simulink model "MotorGenerator1_Component_harness_model"  (R2023a)
settings: Solver=daessc  StartTime=0.0  StopTime=20  RelTol=1e-3  AbsTol=1e-3
PreLoadFcn:
  | MotorGenerator1_Component_harness_setup
undefined symbols (not defined in the file or in its folder): batteryHighVoltage, initial, Minus, motorGenerator1, Plus
libraries: fl_lib x24, nesl_utility x11, sdl_lib x3
settings Model: Creator=isaacito  LastModifiedBy=isaacito
settings SolverCC: AutoScaleAbsTol=off  AlgebraicLoopSolver=TrustRegion
settings OptimizationCC: ReuseModelBlockBuffer=off
settings DebuggingCC: UnconnectedInputMsg=warning  UnconnectedOutputMsg=warning  UnconnectedLineMsg=warning  SymbolicDimsDataTypeCodeGenerationDiagnostic=none
settings ModelReferenceCC: EnableRefExpFcnMdlSchedulingChecks=on
settings SFSimCC: CustomCodeUndefinedFunction=UseInterfaceOnly
settings RTWCC: DLArmComputeVersion=19.05
settings SimscapeCC: SimscapeLogType=all  SimscapeLogSimulationStatistics=on  SimscapeLogLimitData=off  SimscapeLogDataHistory=10000

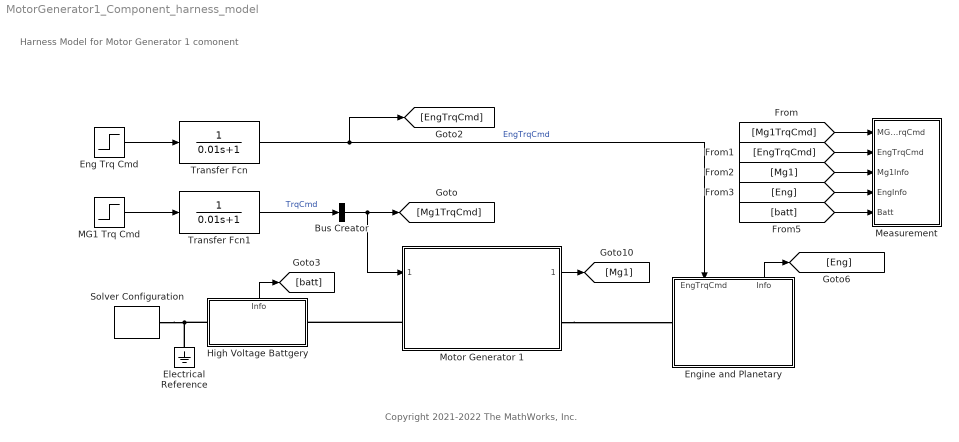
== system MotorGenerator1_Component_harness_model ==
  note: Harness Model for Motor Generator 1 comonent
  note: Copyright 2021-2022 The MathWorks, Inc.
  Bus Creator : BusCreator  Inputs=1
  Electrical Reference : fl_lib/Electrical/Electrical Elements/Electrical Reference
  Eng Trq Cmd : Step  Time=10  Before=100  After=0  SampleTime=0
      settings: AttributesFormatString=|
      | Before %<Before>
      | Time %<Time>
      | After %<After>
  Engine and Planetary : Subsystem
      settings: PortSchema="{\"entries\":[{\"content\":{\"sides\":[{\"content\":{\"connectorIds\":[\"LConn1\"]},\"type\":\"ConnectorPlacement.EquallySpacedRectSide\",\"uuid\":\"98e473f2-6fb6-4bf2-93a0-47b50a56d31a\"},{\"content\":{\"connectorIds\":[],\"side\":\"RIGHT\"},\"type\":\"ConnectorPlacement.EquallySpacedRectSide\",\"uuid\":\"e7c78de6-faab-4a88-b22a-7c9a139264de\"},{\"content\":{\"connectorIds\":[\"In1\",\"Out1\"],\"side\":\"TOP\"},\"type\":\"ConnectorPlacement.EquallySpacedRectSide\",\"uuid\":\"45493563-c3b6-4270-8bd2-a782db83b07f\"}]},\"type\":\"ConnectorPlacement.EquallySpacedConnector\",\"uuid\":\"120a86e3-ef09-4ca7-b56f-7271bd8d5896\"}],\"packageUris\":[\"http://schema.mathworks.com/mf0/Connector/R2020b\"],\"version\":\"1.0\"}"
  High Voltage Battgery : Subsystem
      settings: PortSchema="{\"entries\":[{\"content\":{\"sides\":[{\"content\":{\"connectorIds\":[\"LConn1\"]},\"type\":\"ConnectorPlacement.EquallySpacedRectSide\",\"uuid\":\"8acd7e9a-bb08-4de6-aa14-0989ebba81b9\"},{\"content\":{\"connectorIds\":[\"RConn1\"],\"side\":\"RIGHT\"},\"type\":\"ConnectorPlacement.EquallySpacedRectSide\",\"uuid\":\"f80e1afc-966f-4d6b-84f9-f0b60dd6f20c\"},{\"content\":{\"connectorIds\":[\"Out1\"],\"side\":\"TOP\"},\"type\":\"ConnectorPlacement.EquallySpacedRectSide\",\"uuid\":\"52ccb2b1-bd5e-4dcb-b9b6-0ef03b912c33\"}]},\"type\":\"ConnectorPlacement.EquallySpacedConnector\",\"uuid\":\"b55f48a4-f283-4a77-8513-99b31abb285a\"}],\"packageUris\":[\"http://schema.mathworks.com/mf0/Connector/R2020b\"],\"version\":\"1.0\"}"
  MG1 Trq Cmd : Step  Time=15  After=-5  SampleTime=0
      settings: AttributesFormatString=|
      | Before %<Before>
      | Time %<Time>
      | After %<After>
  Measurement : Subsystem
  Motor Generator 1 : Subsystem  ReferencedSubsystem=MotorDriveUnit_refsub_Basic  torque_max=motorGenerator1.trqMax_Nm  Value=motorGenerator1.powerMax_kW  Tc=motorGenerator1.responseTime_s  eff=motorGenerator1.efficiency_pct  w_eff=motorGenerator1.spd_eff_rpm  T_eff=motorGenerator1.trq_eff_Nm  thermal_mass=motorGenerator1.thermalMass_J_perK  temperature=initial.MG1_Temperature_K  k=motorGenerator1.dampSpringStiffness_Nm_per_rad  mu_visc=motorGenerator1.dampSpringFriction_Nm_per_rpm  w_tol=smoothing.MG1_dampSpringVelTol_rpm  T=initial.MG1_AirTemp_K
      settings: PortSchema="{\"entries\":[{\"content\":{\"sides\":[{\"content\":{\"connectorIds\":[\"In1\",\"LConn1\"]},\"type\":\"ConnectorPlacement.EquallySpacedRectSide\",\"uuid\":\"02d16a10-ccfb-4288-a5a1-1144159c5ca2\"},{\"content\":{\"connectorIds\":[\"Out1\",\"LConn2\"],\"side\":\"RIGHT\"},\"type\":\"ConnectorPlacement.EquallySpacedRectSide\",\"uuid\":\"b2601986-efe5-4f5e-bd54-3f5cb03e9252\"},{\"content\":{\"side\":\"TOP\"},\"type\":\"ConnectorPlacement.EquallySpacedRectSide\",\"uuid\":\"248805f0-4416-4f49-8b0b-c2d3fe77e89e\"}]},\"type\":\"ConnectorPlacement.EquallySpacedConnector\",\"uuid\":\"35449164-35fe-478e-9b2e-66e853caa6da\"}],\"packageUris\":[\"http://schema.mathworks.com/mf0/Connector/R2020b\"],\"version\":\"1.0\"}"
  Solver Configuration : nesl_utility/Solver Configuration  PhysicalDomain=network_engine_domain  SubClassName=solver  LeftPortType=input  RightPortType=generic  Tones=[]  Harmonics=[]  SimulateNoise=off  Profile=off  UseLocalSampling=off  EnableSwitchedLinearOptims=on  FrequencyDomain=off  UseCCode=off  RelTol=0.001  AbsTol=1e-06  MinStep=1e-09  ToWorkspace=off  RevertToSquareIcSolve=off  NumHomotopyIterations=100  PhasorMode=off  PhasorModeNumHarmonics=1  ConsistencySolver=NEWTON_FTOL  IndexReductionMethod=DerivativeReplacement  DoDC=off  ResidualTolerance=1e-09  ConsistencyTolSource=GLOBAL  ConsistencyAbsTol=0.001  ConsistencyRelTol=0.001  ConsistencyTolFactor=0.001  UseLocalSolver=off  LocalSolverChoice=NE_BACKWARD_EULER_ADVANCER  ResolveIndetEquations=on  FunctionEvalNumThread=1  LocalSolverSampleTime=0.001  DoFixedCost=off  MaxNonlinIter=3  MaxModeIter=2  ComputeImpulses=off  ImpulseIterations=2  LinearAlgebra=auto  LinearAlgebraNumThread=0  EquationFormulation=NE_TIME_EF  DelaysMemoryBudget=1024  AutomaticFiltering=on  FilteringTimeConstant=0.001  PartitionStorageMethod=AS_NEEDED  PartitionMemoryBudget=1024  PartitionMethod=ROBUST
      settings: AttributesFormatString=Local solver %<UseLocalSolver>
  Transfer Fcn : TransferFcn  Denominator=[0.01 1]
  Transfer Fcn1 : TransferFcn  Denominator=[0.01 1]
  wires:
  Motor Generator 1/1 -> [Mg1]
  High Voltage Battgery/1(Info) -> [batt]
  Engine and Planetary/1(Info) -> [Eng]
  Eng Trq Cmd/1 -> Transfer Fcn/1
  [Mg1] -> Measurement/3(Mg1Info)
  [Eng] -> Measurement/4(EngInfo)
  [batt] -> Measurement/5(Batt)
  [Mg1TrqCmd] -> Measurement/1(MG1TrqCmd)
  [EngTrqCmd] -> Measurement/2(EngTrqCmd)
  Bus Creator/1 -> Motor Generator 1/1, [Mg1TrqCmd]
  Transfer Fcn/1 -> [EngTrqCmd], Engine and Planetary/1(EngTrqCmd)  "EngTrqCmd"
  Transfer Fcn1/1 -> Bus Creator/1  "TrqCmd"
  MG1 Trq Cmd/1 -> Transfer Fcn1/1
  connections:
  Solver Configuration/RConn1 -- Electrical Reference/LConn1 -- High Voltage Battgery/LConn1
  Motor Generator 1/LConn1 -- High Voltage Battgery/RConn1
  Motor Generator 1/LConn2 -- Engine and Planetary/LConn1

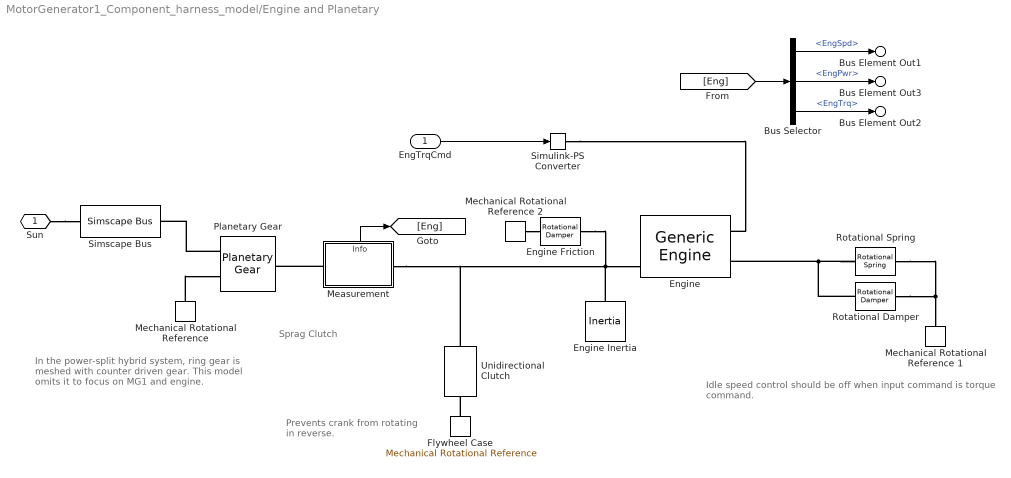
== system MotorGenerator1_Component_harness_model/Engine and Planetary ==
  note: Idle speed control should be off
      | when input command is torque command.
  note: Prevents crank from
      | rotating in reverse.
  note: In the power-split hybrid system,
      | ring gear is meshed with
      | counter driven gear.
      | This model omits it to focus on
      | MG1 and engine.
  note: Sprag Clutch
  EngTrqCmd : Inport
  Bus Selector : BusSelector  OutputSignals=EngSpd,EngPwr,EngTrq
  Engine : sdl_lib/Engines & Motors/Generic Engine  input_type=sdl.enum.GenericEngineInputType.TorqueCommand  model_parameterization=sdl.enum.engineParameterization.polynomial  engine_type=sdl.enum.engineType.Generic  Trq_max=145 N*m  w_Trq_max=3500 rpm  P_max=75 kW  w_P_max=7500 rpm  w_max=7000 rpm  w_min=500 rpm  w_tab=[500, 1000, 2000, 3000, 4300, 5000, 6000, 7000] rpm  trq_tab=[250, 280, 330, 360, 380, 370, 350, 310] N*m  pwr_tab=[10, 30, 70, 110, 165, 190, 220, 230] kW  interp_method=simscape.enum.interpolation.linear  w_thr=100 rpm  model_inertia=sdl.enum.model_inertia.off  inertia=1 kg*m^2  initial_velocity=800 rpm  model_time_constant=sdl.enum.lagOffOn.on  time_constant=0.1 s  initial_normalized_throttle=0  fc_model=sdl.enum.fuel_consumption_model.FuelOff  fc_per_rev=25 mg/rev  fc_w_tab=[1000, 2000, 3000, 4000, 5000, 6000] rpm  fc_trq_tab=[0, 80, 160, 200, 240, 320, 360, 400] N*m  fc_tab=[.5, .9, 1.4, 1.6, 1.9, 2.7, 3.4, 4.4; 1, 1.7, 2.7, 3.1, 3.6, 5, 6, 7.4; 1.4, 2.7, 4, 4.8, 5.6, 7.5, 8.5, 10.5; 2, 3.6, 5.8, 6.7, 8, 10.4, 11.7, 13.3; 2.5, 4.8, 7.9, 9.4, 10.8, 14, 16.2, 18.6; 3.1, 6, 10.3, 11.9, 13.8, 18.4, 22, 26.5] g/s  bmep_tab=[0, 250, 500, 625, 750, 1000, 1150, 1250] kPa  bsfc_tab=[410, 380, 300, 280, 270, 290, 320, 380; 410, 370, 290, 270, 260, 270, 285, 320; 415, 380, 290, 275, 265, 270, 270, 300; 420, 390, 310, 290, 285, 280, 280, 285; 430, 410, 340, 320, 310, 300, 310, 320; 450, 430, 370, 340, 330, 330, 350, 380] g/(hr*kW)  fc_interp_method=simscape.enum.interpolation.linear  displaced_volume=400 cm^3  rev_per_cycle=2  idle_speed=false  idle_speed_reference=1000 rpm  tau_controller=0.1 s  idle_w_thr=1 rpm  redline=false  redline_speed=5000 rpm  tau_redline=1 s  redline_w_thr=1 rpm
      settings: InternalSimscapePortConfiguration="{\"Bottom\":[],\"Left\":[{\"id\":\"TrqCmd\",\"label\":\"Trq\",\"type\":\"input\"},{\"id\":\"B\",\"label\":\"B\",\"type\":\"foundation.mechanical.rotational.rotational\"}],\"Right\":[{\"id\":\"P\",\"label\":\"P\",\"type\":\"output\"},{\"id\":\"FC\",\"label\":\"FC\",\"type\":\"output\"},{\"id\":\"F\",\"label\":\"F\",\"type\":\"foundation.mechanical.rotational.rotational\"}],\"Top\":[]}"
  Engine Friction : fl_lib/Mechanical/Rotational Elements/Rotational Damper  D=0.02 m*N/rpm  w_specify=off  w_priority=None  w=0 rad/s  w_nominal_specify=off  w_nominal_unit=rad/s  w_nominal_value=1  t_specify=off  t_priority=None  t=0 N*m  t_nominal_specify=off  t_nominal_unit=N*m  t_nominal_value=1
  Engine Inertia : fl_lib/Mechanical/Rotational Elements/Inertia  inertia=0.02 kg*m^2  num_ports=foundation.enum.numPorts2.one  w_specify=on  w_priority=High  w=initial.engine_speed_rpm rpm  w_nominal_specify=off  w_nominal_unit=rad/s  w_nominal_value=1  t_specify=off  t_priority=None  t=0 N*m  t_nominal_specify=off  t_nominal_unit=N*m  t_nominal_value=1
      settings: AttributesFormatString=|
      | %<inertia> (%<inertia_unit>)
      | %<w> (%<w_unit>)
      | Priority: %<w_priority>
  Flywheel Case : fl_lib/Mechanical/Rotational Elements/Mechanical Rotational Reference
  Measurement : Subsystem
      settings: PortSchema="{\"entries\":[{\"content\":{\"sides\":[{\"content\":{\"connectorIds\":[\"LConn1\"]},\"type\":\"ConnectorPlacement.EquallySpacedRectSide\",\"uuid\":\"98e473f2-6fb6-4bf2-93a0-47b50a56d31a\"},{\"content\":{\"connectorIds\":[\"RConn1\"],\"side\":\"RIGHT\"},\"type\":\"ConnectorPlacement.EquallySpacedRectSide\",\"uuid\":\"e7c78de6-faab-4a88-b22a-7c9a139264de\"},{\"content\":{\"connectorIds\":[\"Out1\"],\"side\":\"TOP\"},\"type\":\"ConnectorPlacement.EquallySpacedRectSide\",\"uuid\":\"45493563-c3b6-4270-8bd2-a782db83b07f\"}]},\"type\":\"ConnectorPlacement.EquallySpacedConnector\",\"uuid\":\"120a86e3-ef09-4ca7-b56f-7271bd8d5896\"}],\"packageUris\":[\"http://schema.mathworks.com/mf0/Connector/R2020b\"],\"version\":\"1.0\"}"
  Mechanical Rotational Reference : fl_lib/Mechanical/Rotational Elements/Mechanical Rotational Reference
  Mechanical Rotational Reference 1 : fl_lib/Mechanical/Rotational Elements/Mechanical Rotational Reference
  Mechanical Rotational Reference 2 : fl_lib/Mechanical/Rotational Elements/Mechanical Rotational Reference
  Planetary Gear : sdl_lib/Gears/Planetary Gear  rs_ratio=78/30  friction_model=sdl.enum.gear_friction.constant  efficiency=[0.98 0.98]  temperature_TLU=[280, 300, 320] K  efficiency_sp_TLU=[.95, .9, .85]  efficiency_rp_TLU=[.95, .9, .85]  pwr_thr=[10 10] W  mu_visc=[0.001 0.001] m*N/rpm  model_inertia=simscape.enum.onoff.on  planet_inertia=0.001 kg*m^2  thermal_mass=50 J/K  T_init=300 K
  Rotational Damper : fl_lib/Mechanical/Rotational Elements/Rotational Damper  D=100 kN*m/rpm  w_specify=off  w_priority=None  w=0 rad/s  w_nominal_specify=off  w_nominal_unit=rad/s  w_nominal_value=1  t_specify=off  t_priority=None  t=0 N*m  t_nominal_specify=off  t_nominal_unit=N*m  t_nominal_value=1
  Rotational Spring : fl_lib/Mechanical/Rotational Elements/Rotational Spring  spr_rate=1 kN*m/rad  w_specify=off  w_priority=None  w=0 rad/s  w_nominal_specify=off  w_nominal_unit=rad/s  w_nominal_value=1  t_specify=off  t_priority=None  t=0 N*m  t_nominal_specify=off  t_nominal_unit=N*m  t_nominal_value=1  phi_specify=on  phi_priority=Low  phi=0 rad  phi_nominal_specify=off  phi_nominal_unit=rad  phi_nominal_value=1
      settings: AttributesFormatString=Deformation priority: %<phi_priority>
  Simscape Bus : SimscapeBus  HierarchyStrings=AngSpd  ConnectionType=Bus: Bus_Rotational
  Simulink-PS Converter : nesl_utility/Simulink-PS Converter  PhysicalDomain=network_engine_domain  SubClassName=ps_input  LeftPortType=input  RightPortType=output  PseudoPeriodic=off  Frequencies=[]  NoiseDistribution=none  NoiseParameters=[]  Unit=N*m  AffineConversion=off  FilteringAndDerivatives=provide  SimscapeFilterOrder=1  InputFilterTimeConstant=0.001  UdotUserProvided=0
  Unidirectional Clutch : sdl_lib/Clutches/Unidirectional Clutch  transmission_direction=2  initial_state_locked=sdl.enum.initial_lock.unlocked
      settings: AttributesFormatString=%<initial_state_locked>  InternalSimscapePortConfiguration="{\"Bottom\":[],\"Left\":[{\"id\":\"H\",\"label\":\"H\",\"type\":\"foundation.mechanical.rotational.rotational\"}],\"Right\":[{\"id\":\"R\",\"label\":\"R\",\"type\":\"foundation.mechanical.rotational.rotational\"}],\"Top\":[]}"
  Sun : PMIOPort  Side=Left
  Bus Element Out1 : Outport  PortName=Info  Element=EngSpd
      settings: AttributesFormatString=%<Unit>
  Bus Element Out3 : Outport  PortName=Info  Element=EngPwr
      settings: AttributesFormatString=%<Unit>
  Bus Element Out2 : Outport  PortName=Info  Element=EngTrq
      settings: AttributesFormatString=%<Unit>
  wires:
  Measurement/1(Info) -> [Eng]
  [Eng] -> Bus Selector/1
  Bus Selector/1 -> Bus Element Out1/1  "<EngSpd>"
  Bus Selector/2 -> Bus Element Out3/1  "<EngPwr>"
  Bus Selector/3 -> Bus Element Out2/1  "<EngTrq>"
  EngTrqCmd/1 -> Simulink-PS Converter/1
  connections:
  Planetary Gear/RConn2 -- Simscape Bus/LConn1
  Sun/RConn1 -- Simscape Bus/RConn1
  Flywheel Case/LConn1 -- Unidirectional Clutch/RConn1
  Rotational Spring/RConn1 -- Rotational Damper/RConn1 -- Mechanical Rotational Reference 1/LConn1
  Rotational Spring/LConn1 -- Engine/LConn2 -- Rotational Damper/LConn1
  Mechanical Rotational Reference 2/LConn1 -- Engine Friction/RConn1
  Engine Friction/LConn1 -- Unidirectional Clutch/LConn1 -- Measurement/RConn1 -- Engine Inertia/LConn1 -- Engine/RConn3
  Measurement/LConn1 -- Planetary Gear/LConn1
  Mechanical Rotational Reference/LConn1 -- Planetary Gear/RConn1
  Simulink-PS Converter/RConn1 -- Engine/LConn1

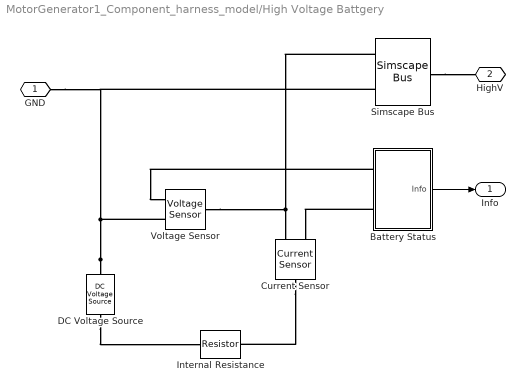
== system MotorGenerator1_Component_harness_model/High Voltage Battgery ==
  Battery Status : Subsystem
  Current Sensor : fl_lib/Electrical/Electrical Sensors/Current Sensor
  DC Voltage Source : fl_lib/Electrical/Electrical Sources/DC Voltage Source  v0=batteryHighVoltage.voltage_V V
      settings: AttributesFormatString=%<v0> [%<v0_unit>]
  Internal Resistance : fl_lib/Electrical/Electrical Elements/Resistor  R=batteryHighVoltage.internal_R_Ohm Ohm  i_specify=off  i_priority=High  i=0 A  i_nominal_specify=off  i_nominal_unit=A  i_nominal_value=1  v_specify=off  v_priority=High  v=0 V  v_nominal_specify=off  v_nominal_unit=V  v_nominal_value=1
      settings: AttributesFormatString=%<R> [%<R_unit>]
  Simscape Bus : SimscapeBus  HierarchyStrings=Plus;Minus  ConnectionType=Bus: Bus_HighVoltage
      settings: AttributesFormatString=%<ConnectionType>
  Voltage Sensor : fl_lib/Electrical/Electrical Sensors/Voltage Sensor
  GND : PMIOPort  Side=Left
  HighV : PMIOPort  Port=2  Side=Right
  Info : Outport
  wires:
  Battery Status/1(Info) -> Info/1
  connections:
  DC Voltage Source/RConn1 -- Simscape Bus/LConn2 -- GND/RConn1 -- Voltage Sensor/RConn2
  Simscape Bus/LConn1 -- Voltage Sensor/LConn1 -- Current Sensor/RConn2
  Battery Status/LConn2 -- Current Sensor/RConn1
  Simscape Bus/RConn1 -- HighV/RConn1
  Current Sensor/LConn1 -- Internal Resistance/RConn1
  DC Voltage Source/LConn1 -- Internal Resistance/LConn1
  Battery Status/LConn1 -- Voltage Sensor/RConn1

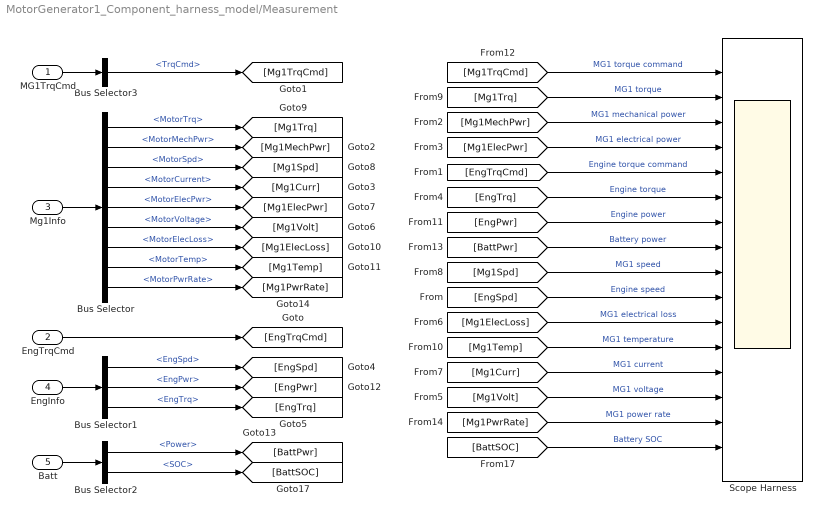
== system MotorGenerator1_Component_harness_model/Measurement ==
  MG1TrqCmd : Inport
  EngTrqCmd : Inport  Port=2
  Mg1Info : Inport  Port=3
  EngInfo : Inport  Port=4
  Batt : Inport  Port=5
  Bus Selector : BusSelector  OutputSignals=MotorTrq,MotorMechPwr,MotorSpd,MotorCurrent,MotorElecPwr,MotorVoltage,MotorElecLoss,MotorTemp,MotorPwrRate
  Bus Selector1 : BusSelector  OutputSignals=EngSpd,EngPwr,EngTrq
  Bus Selector2 : BusSelector  OutputSignals=Power,SOC
  Bus Selector3 : BusSelector  OutputSignals=TrqCmd
  Scope Harness : Scope  NumInputPorts=16
  wires:
  EngInfo/1 -> Bus Selector1/1
  Mg1Info/1 -> Bus Selector/1
  EngTrqCmd/1 -> [EngTrqCmd]
  Batt/1 -> Bus Selector2/1
  Bus Selector/1 -> [Mg1Trq]  "<MotorTrq>"
  Bus Selector/2 -> [Mg1MechPwr]  "<MotorMechPwr>"
  Bus Selector/3 -> [Mg1Spd]  "<MotorSpd>"
  Bus Selector/4 -> [Mg1Curr]  "<MotorCurrent>"
  Bus Selector/5 -> [Mg1ElecPwr]  "<MotorElecPwr>"
  Bus Selector/6 -> [Mg1Volt]  "<MotorVoltage>"
  Bus Selector/7 -> [Mg1ElecLoss]  "<MotorElecLoss>"
  Bus Selector/8 -> [Mg1Temp]  "<MotorTemp>"
  Bus Selector1/1 -> [EngSpd]  "<EngSpd>"
  Bus Selector1/2 -> [EngPwr]  "<EngPwr>"
  Bus Selector1/3 -> [EngTrq]  "<EngTrq>"
  Bus Selector2/1 -> [BattPwr]  "<Power>"
  Bus Selector2/2 -> [BattSOC]  "<SOC>"
  [Mg1TrqCmd] -> Scope Harness/1  "MG1 torque command"
  [Mg1Trq] -> Scope Harness/2  "MG1 torque"
  [Mg1MechPwr] -> Scope Harness/3  "MG1 mechanical power"
  [Mg1ElecPwr] -> Scope Harness/4  "MG1 electrical power"
  [EngTrqCmd] -> Scope Harness/5  "Engine torque command"
  [EngTrq] -> Scope Harness/6  "Engine torque"
  [EngPwr] -> Scope Harness/7  "Engine power"
  [BattPwr] -> Scope Harness/8  "Battery power"
  [Mg1Spd] -> Scope Harness/9  "MG1 speed"
  [EngSpd] -> Scope Harness/10  "Engine speed"
  [Mg1ElecLoss] -> Scope Harness/11  "MG1 electrical loss"
  [Mg1Temp] -> Scope Harness/12  "MG1 temperature"
  [Mg1Curr] -> Scope Harness/13  "MG1 current"
  [Mg1Volt] -> Scope Harness/14  "MG1 voltage"
  [BattSOC] -> Scope Harness/16  "Battery SOC"
  MG1TrqCmd/1 -> Bus Selector3/1
  Bus Selector3/1 -> [Mg1TrqCmd]  "<TrqCmd>"
  Bus Selector/9 -> [Mg1PwrRate]  "<MotorPwrRate>"
  [Mg1PwrRate] -> Scope Harness/15  "MG1 power rate"

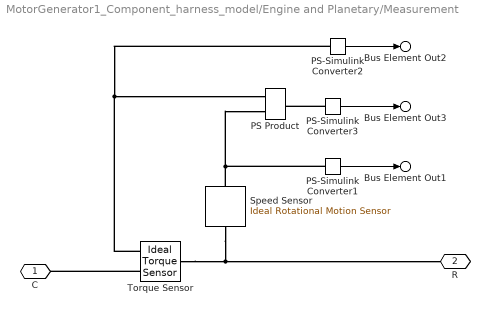
== system MotorGenerator1_Component_harness_model/Engine and Planetary/Measurement ==
  PS Product : fl_lib/Physical Signals/Functions/PS Product
  PS-Simulink Converter1 : nesl_utility/PS-Simulink Converter  PhysicalDomain=network_engine_domain  SubClassName=ps_output  LeftPortType=input  RightPortType=output  PseudoPeriodic=off  Frequencies=[]  VectorFormat=1-D array  Unit=rpm  AffineConversion=off
  PS-Simulink Converter2 : nesl_utility/PS-Simulink Converter  PhysicalDomain=network_engine_domain  SubClassName=ps_output  LeftPortType=input  RightPortType=output  PseudoPeriodic=off  Frequencies=[]  VectorFormat=1-D array  Unit=N*m  AffineConversion=off
  PS-Simulink Converter3 : nesl_utility/PS-Simulink Converter  PhysicalDomain=network_engine_domain  SubClassName=ps_output  LeftPortType=input  RightPortType=output  PseudoPeriodic=off  Frequencies=[]  VectorFormat=1-D array  Unit=kW  AffineConversion=off
  Speed Sensor : fl_lib/Mechanical/Mechanical Sensors/Ideal Rotational Motion Sensor  reference=foundation.enum.MeasurementReference.absolute  acceleration_port=false  velocity_port=true  position_port=false  wrap_angle=false  offset=0 rad
      settings: InternalSimscapePortConfiguration="{\"Bottom\":[],\"Left\":[{\"id\":\"R\",\"label\":\"R\",\"type\":\"foundation.mechanical.rotational.rotational\"}],\"Right\":[{\"id\":\"W\",\"label\":\"W\",\"type\":\"output\"}],\"Top\":[]}"
  Torque Sensor : fl_lib/Mechanical/Mechanical Sensors/Ideal Torque Sensor
  C : PMIOPort  Side=Left
  R : PMIOPort  Port=2  Side=Right
  Bus Element Out1 : Outport  PortName=Info  Element=EngSpd
      settings: AttributesFormatString=%<Unit>
  Bus Element Out3 : Outport  PortName=Info  Element=EngPwr
      settings: AttributesFormatString=%<Unit>
  Bus Element Out2 : Outport  PortName=Info  Element=EngTrq
      settings: AttributesFormatString=%<Unit>
  wires:
  PS-Simulink Converter2/1 -> Bus Element Out2/1
  PS-Simulink Converter3/1 -> Bus Element Out3/1
  PS-Simulink Converter1/1 -> Bus Element Out1/1
  connections:
  Torque Sensor/RConn1 -- C/RConn1
  Speed Sensor/RConn1 -- PS-Simulink Converter1/LConn1 -- PS Product/LConn2
  PS-Simulink Converter3/LConn1 -- PS Product/RConn1
  Torque Sensor/RConn2 -- PS-Simulink Converter2/LConn1 -- PS Product/LConn1
  Torque Sensor/LConn1 -- R/RConn1 -- Speed Sensor/LConn1

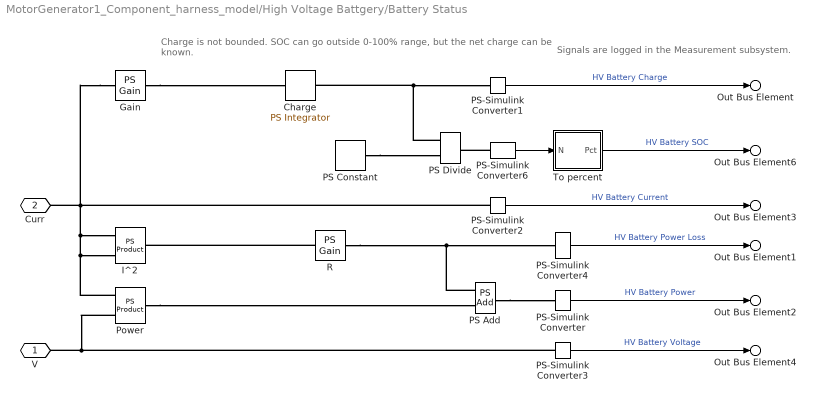
== system MotorGenerator1_Component_harness_model/High Voltage Battgery/Battery Status ==
  note: Signals are logged in the Measurement subsystem.
  note: Charge is not bounded. SOC can go outside 0-100% range,
      | but the net charge can be known.
  Charge : fl_lib/Physical Signals/Linear Operators/PS Integrator  reset_method=foundation.enum.IntegratorResetSpec.None  initial_condition_spec=foundation.enum.IntegratorICSpec.Internal  saturation_spec=foundation.enum.IntegratorSaturationSpec.None  saturation_source_spec=foundation.enum.IntegratorSaturationSourceSpec.Internal  x0=initial.hvBattery_Charge_Ahr A*hr  xu=inf s  xl=-inf s
      settings: AttributesFormatString=%<x0> [%<x0_unit>]
  Gain : fl_lib/Physical Signals/Functions/PS Gain  gain=-1
      settings: AttributesFormatString=%<gain>
  I^2 : fl_lib/Physical Signals/Functions/PS Product
  PS Add : fl_lib/Physical Signals/Functions/PS Add
  PS Constant : fl_lib/Physical Signals/Sources/PS Constant  constant=batteryHighVoltage.charge_Ahr A*hr
      settings: AttributesFormatString=%<constant> [%<constant_unit>]
  PS Divide : fl_lib/Physical Signals/Functions/PS Divide
  PS-Simulink Converter : nesl_utility/PS-Simulink Converter  PhysicalDomain=network_engine_domain  SubClassName=ps_output  LeftPortType=input  RightPortType=output  PseudoPeriodic=off  Frequencies=[]  VectorFormat=1-D array  Unit=kW  AffineConversion=off
  PS-Simulink Converter1 : nesl_utility/PS-Simulink Converter  PhysicalDomain=network_engine_domain  SubClassName=ps_output  LeftPortType=input  RightPortType=output  PseudoPeriodic=off  Frequencies=[]  VectorFormat=1-D array  Unit=A*hr  AffineConversion=off
  PS-Simulink Converter2 : nesl_utility/PS-Simulink Converter  PhysicalDomain=network_engine_domain  SubClassName=ps_output  LeftPortType=input  RightPortType=output  PseudoPeriodic=off  Frequencies=[]  VectorFormat=1-D array  Unit=A  AffineConversion=off
  PS-Simulink Converter3 : nesl_utility/PS-Simulink Converter  PhysicalDomain=network_engine_domain  SubClassName=ps_output  LeftPortType=input  RightPortType=output  PseudoPeriodic=off  Frequencies=[]  VectorFormat=1-D array  Unit=V  AffineConversion=off
  PS-Simulink Converter4 : nesl_utility/PS-Simulink Converter  PhysicalDomain=network_engine_domain  SubClassName=ps_output  LeftPortType=input  RightPortType=output  PseudoPeriodic=off  Frequencies=[]  VectorFormat=1-D array  Unit=W  AffineConversion=off
  PS-Simulink Converter6 : nesl_utility/PS-Simulink Converter  PhysicalDomain=network_engine_domain  SubClassName=ps_output  LeftPortType=input  RightPortType=output  PseudoPeriodic=off  Frequencies=[]  VectorFormat=1-D array  Unit=1  AffineConversion=off
  Power : fl_lib/Physical Signals/Functions/PS Product
  R : fl_lib/Physical Signals/Functions/PS Gain  gain=batteryHighVoltage.internal_R_Ohm Ohm
      settings: AttributesFormatString=%<gain> [%<gain_unit>]
  To percent : Subsystem
  V : PMIOPort  Side=Left
  Curr : PMIOPort  Port=2  Side=Left
  Out Bus Element : Outport  PortName=Info  Element=Charge
      settings: AttributesFormatString=%<Unit>
  Out Bus Element3 : Outport  PortName=Info  Element=Current
      settings: AttributesFormatString=%<Unit>
  Out Bus Element1 : Outport  PortName=Info  Element=PowerLoss
      settings: AttributesFormatString=%<Unit>
  Out Bus Element2 : Outport  PortName=Info  Element=Power
      settings: AttributesFormatString=%<Unit>
  Out Bus Element4 : Outport  PortName=Info  Element=Voltage
      settings: AttributesFormatString=%<Unit>
  Out Bus Element6 : Outport  PortName=Info  Element=SOC
      settings: AttributesFormatString=%<Unit>
  wires:
  PS-Simulink Converter6/1 -> To percent/1(N)
  To percent/1(Pct) -> Out Bus Element6/1  "HV Battery SOC"
  PS-Simulink Converter3/1 -> Out Bus Element4/1  "HV Battery Voltage"
  PS-Simulink Converter2/1 -> Out Bus Element3/1  "HV Battery Current"
  PS-Simulink Converter4/1 -> Out Bus Element1/1  "HV Battery Power Loss"
  PS-Simulink Converter1/1 -> Out Bus Element/1  "HV Battery Charge"
  PS-Simulink Converter/1 -> Out Bus Element2/1  "HV Battery Power"
  connections:
  PS-Simulink Converter6/LConn1 -- PS Divide/RConn1
  Power/RConn1 -- PS Add/LConn2
  PS Constant/RConn1 -- PS Divide/LConn2
  PS Add/RConn1 -- PS-Simulink Converter/LConn1
  R/LConn1 -- I^2/RConn1
  PS Divide/LConn1 -- PS-Simulink Converter1/LConn1 -- Charge/RConn1
  Gain/RConn1 -- Charge/LConn1
  PS Add/LConn1 -- PS-Simulink Converter4/LConn1 -- R/RConn1
  Power/LConn1 -- PS-Simulink Converter3/LConn1 -- V/RConn1
  Gain/LConn1 -- PS-Simulink Converter2/LConn1 -- Curr/RConn1 -- I^2/LConn1 -- Power/LConn2 -- I^2/LConn2

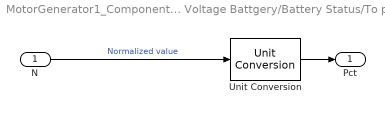
== system MotorGenerator1_Component_harness_model/High Voltage Battgery/Battery Status/To percent ==
  N : Inport
  Unit Conversion : UnitConversion
  Pct : Outport  Unit=%
      settings: AttributesFormatString=%<Unit>
  wires:
  N/1 -> Unit Conversion/1  "Normalized value"
  Unit Conversion/1 -> Pct/1
